simulink model "Sim_BPSK_4"  (Simulink 10.1)
settings: Solver=VariableStepAuto  StartTime=0.0  StopTime=100000  RelTol=1e-3
libraries: commdigbbndpm3 x2, commchan3 x1, commsink2 x1, commrandsrc2 x1
settings Model: LogicAnalyzerSignalOrdering=78ef603b-b1d8-47e3-8577-e9d9a9fadcef,add060ce-72b2-4865-9060-7dfe855c1b3d  Creator=mawenjian  LastModifiedBy=mawenjian
settings DataIOCC: SaveFormat=Dataset  ReturnWorkspaceOutputs=on
settings OptimizationCC: LifeSpan=auto
settings DebuggingCC: UnderspecifiedInitializationDetection=Simplified  MergeDetectMultiDrivingBlocksExec=error  SFUnexpectedBacktrackingDiag=error  SFNoUnconditionalDefaultTransitionDiag=error  SFExecutionAtInitializationDiag=warning  ArithmeticOperatorsInVariantConditions=error
settings HardwareCC: ProdBitPerPointer=64  ProdBitPerSizeT=64  ProdBitPerPtrDiffT=64  ProdLargestAtomicFloat=Float  ProdIntDivRoundTo=Zero  ProdEndianess=LittleEndian  ProdWordSize=64  ProdHWDeviceType=Intel->x86-64 (Windows64)
settings ModelReferenceCC: PropagateSignalLabelsOutOfModel=on
settings SFSimCC: SimUseLocalCustomCode=on  CustomCodeUndefinedFunction=FilterOut
settings RTWCC: RTWUseLocalCustomCode=on
settings CodeAppCC: StateflowObjectComments=off
settings GRTTargetCC: TargetLangStandard=C99 (ISO)  CombineOutputUpdateFcns=on  GRTInterface=off
settings ConfigComp: CovMetricSettings=dwe  CovHtmlReporting=off  CovSaveCumulativeToWorkspaceVar=off  CovSaveSingleToWorkspaceVar=off  CovExternalEMLEnable=on

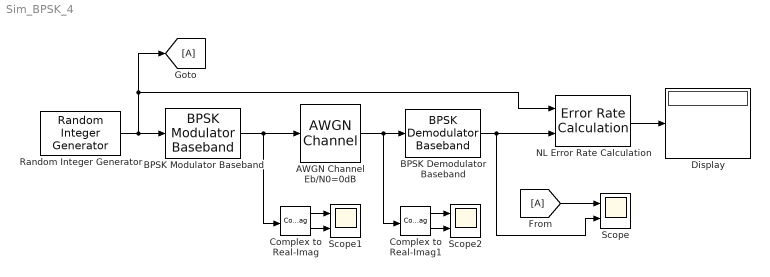
== system Sim_BPSK_4 ==
  AWGN Channel Eb/N0=0dB : commchan3/AWGN Channel  InputProcessing=Columns as channels (frame based)  seed=67  noiseMode="Signal to noise ratio  (Eb/No)"  EbNodB=0  EsNodB=4  SNRdB=10  bitsPerSym=1  Ps=1  Tsym=1  variance=1
  BPSK Demodulator Baseband : commdigbbndpm3/BPSK Demodulator Baseband  DecType=Hard decision  VarSource=Dialog  Variance=1  Ph=0  outDtype=Inherit via internal rule  derotateFactorWordLen=2  derotateFactorDataTypeStr=Inherit: Same word length as input  derotateFactorLastDataTypeStr=Inherit: Same word length as input
  BPSK Modulator Baseband : commdigbbndpm3/BPSK Modulator Baseband  Ph=0  outDtype=double  outWordLen=16  outUDDataType=sfix(16)  outFracLenMode=Best precision  outFracLen=15  outDataTypeStr=double  outLastDataTypeStr=double
  Complex to Real-Imag : ComplexToRealImag
  Complex to Real-Imag1 : ComplexToRealImag
  Display : Display
  NL Error Rate Calculation : commsink2/Error Rate Calculation  N=0  st_delay=0  cp_mode=Entire frame  subframe=[]  PMode=Port  WsName=ErrorVec  RsMode2=off  stop=off  numErr=100  maxBits=1e6
  Random Integer Generator : commrandsrc2/Random Integer Generator  mul=2  seed=37  Ts=1  frameBased=off  sampPerFrame=1000  orient=off  outDataType=double
      settings: SourceProductBaseCode=CM
  Scope : Scope  NumInputPorts=2
  Scope1 : Scope  NumInputPorts=2
  Scope2 : Scope  NumInputPorts=2
  wires:
  Random Integer Generator/1 -> NL Error Rate Calculation/1, [A], BPSK Modulator Baseband/1
  BPSK Modulator Baseband/1 -> Complex to Real-Imag/1, AWGN Channel Eb/N0=0dB/1
  AWGN Channel Eb/N0=0dB/1 -> BPSK Demodulator Baseband/1, Complex to Real-Imag1/1
  BPSK Demodulator Baseband/1 -> NL Error Rate Calculation/2, Scope/2
  Complex to Real-Imag/1 -> Scope1/1
  Complex to Real-Imag/2 -> Scope1/2
  Complex to Real-Imag1/1 -> Scope2/1
  Complex to Real-Imag1/2 -> Scope2/2
  NL Error Rate Calculation/1 -> Display/1
  [A] -> Scope/1
